simulink model "system_continuous"  (R2026b)
settings: Solver=VariableStepAuto  StopTime=20
values from neighbouring files (symbols this model uses):
  A_sys = zeros(14, 14)    [controller_observer_design.m]    (also in setup.m)
  B_sys = zeros(14, 4)    [controller_observer_design.m]    (also in setup.m)
  C_sys = zeros(6, 14)    [controller_observer_design.m]    (also in setup.m)
  K = lqr(A_sys, B_sys, Q, R)    [controller_observer_design.m]    (also in setup.m)
  omega2u = [k, k, k, k; L*k, 0, -L*k, 0; 0, L*k, 0, -L*k; b, -b, b, -b]    [controller_observer_design.m]    (also in notes.m; setup.m)
  parameters =     [parameters.mat]
  u2omega = (1/(4*b*L*k)) * [b*L, 2*b, 0, L*k; b*L, 0, 2*b, -L*k; b*L, -2*b, 0, L*k; b*L, 0, -2*b, -L*k]    [controller_observer_design.m]    (also in notes.m; setup.m)
undefined symbols (not defined in the file or in its folder): L_obs
settings Model: Creator=elton  LastModifiedBy=elton

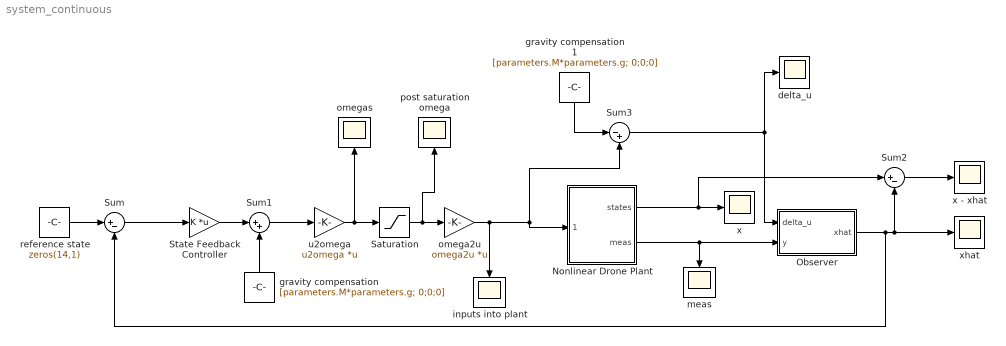
== system system_continuous ==
  Nonlinear Drone Plant : Subsystem
  Observer : Subsystem
  Saturation : Saturate  UpperLimit=250000  LowerLimit=-250000
  State Feedback Controller : Gain  Gain=K  Multiplication=Matrix(K*u)
  Sum : Sum  Inputs=|+-
  Sum1 : Sum  Inputs=|++
  Sum2 : Sum  Inputs=|+-
  Sum3 : Sum  Inputs=|-+
  delta_u : Scope
      settings: ActiveDisplayYMinimum=-0.1401923631580794  ActiveDisplayYMaximum=0.1652403175832419
  gravity compensation : Constant  Value=[parameters.M*parameters.g; 0;0;0]
  gravity compensation1 : Constant  Value=[parameters.M*parameters.g; 0;0;0]
  inputs into plant : Scope
      settings: ActiveDisplayYMinimum=-2.3883084159431922  ActiveDisplayYMaximum=20.39828479264926  DataLoggingVariableName=ScopeData7
  meas : Scope
      settings: ActiveDisplayYMinimum=-955.77756320006051  ActiveDisplayYMaximum=3490.5526217286788
  omega2u : Gain  Gain=omega2u  Multiplication=Matrix(K*u)
  omegas : Scope
      settings: ActiveDisplayYMinimum=-2.059012913011611E+9  ActiveDisplayYMaximum=2.4856689660528789E+9  DataLoggingVariableName=ScopeData8
  post saturation omega : Scope
      settings: ActiveDisplayYMinimum=126867.29383047414  ActiveDisplayYMaximum=168019.94398868005  DataLoggingVariableName=ScopeData9
  reference state : Constant  Value=zeros(14,1)
  u2omega : Gain  Gain=u2omega  Multiplication=Matrix(K*u)
  x : Scope
      settings: ActiveDisplayYMinimum=-2.6435151573110338  ActiveDisplayYMaximum=2.3244072174192603  DataLoggingVariableName=ScopeData6
  x - xhat : Scope
      settings: ActiveDisplayYMinimum=-0.31631682024418123  ActiveDisplayYMaximum=0.17275572014351576  DataLoggingVariableName=ScopeData2
  xhat : Scope
      settings: ActiveDisplayYMinimum=-2.6439782880906106  ActiveDisplayYMaximum=2.3281571087039121  DataLoggingVariableName=ScopeData3
  wires:
  omega2u/1 -> Sum3/2, Nonlinear Drone Plant/1(inputs), inputs into plant/1
  Nonlinear Drone Plant/1(states) -> x/1, Sum2/1
  Sum2/1 -> x - xhat/1
  Sum/1 -> State Feedback Controller/1
  gravity compensation1/1 -> Sum3/1
  reference state/1 -> Sum/1
  gravity compensation/1 -> Sum1/2
  Observer/1(xhat) -> xhat/1, Sum2/2, Sum/2
  u2omega/1 -> Saturation/1, omegas/1
  Saturation/1 -> post saturation omega/1, omega2u/1
  State Feedback Controller/1 -> Sum1/1
  Sum3/1 -> delta_u/1, Observer/1(delta_u)
  Sum1/1 -> u2omega/1
  Nonlinear Drone Plant/2(meas) -> Observer/2(y), meas/1

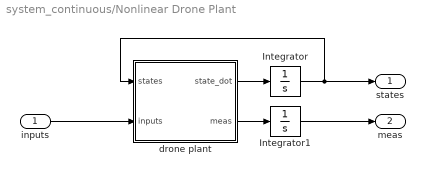
== system system_continuous/Nonlinear Drone Plant ==
  inputs : Inport
  Integrator : Integrator  InitialCondition=[zeros(12,1);0.05;0]
  Integrator1 : Integrator
  drone plant : MATLAB Function  TreatAsAtomicUnit=on
  states : Outport
  meas : Outport  Port=2
  wires:
  drone plant/1(state_dot) -> Integrator/1
  Integrator/1 -> states/1, drone plant/1(states)
  inputs/1 -> drone plant/2(inputs)
  Integrator1/1 -> meas/1
  drone plant/2(meas) -> Integrator1/1

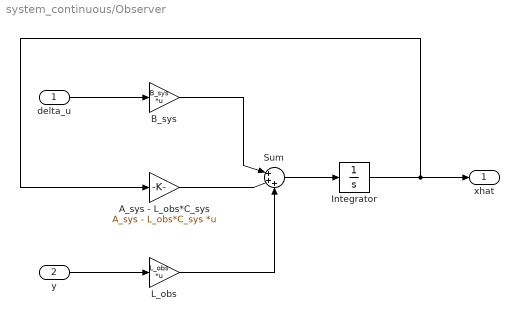
== system system_continuous/Observer ==
  delta_u : Inport
  y : Inport  Port=2
  A_sys - L_obs*C_sys : Gain  Gain=A_sys - L_obs*C_sys  Multiplication=Matrix(K*u)
  B_sys : Gain  Gain=B_sys  Multiplication=Matrix(K*u)
  Integrator : Integrator
  L_obs : Gain  Gain=L_obs  Multiplication=Matrix(K*u)
  Sum : Sum  Inputs=|+++
  xhat : Outport
  wires:
  y/1 -> L_obs/1
  B_sys/1 -> Sum/1
  L_obs/1 -> Sum/3
  A_sys - L_obs*C_sys/1 -> Sum/2
  Sum/1 -> Integrator/1
  Integrator/1 -> A_sys - L_obs*C_sys/1, xhat/1
  delta_u/1 -> B_sys/1

== matlab function system_continuous/Nonlinear Drone Plant/drone plant ==
  data: states input size=14; inputs input size=4; state_dot output size=14; parameters parameter; meas output
%% non-linear state space
function [state_dot, meas]  = nonlin_state_space(states, inputs, parameters)
m     = parameters.m;
m_p    = parameters.m_p;
M     = m + m_p;
g     = parameters.g;
l     = parameters.l;
k_D    = parameters.k_D;
I_xx  = parameters.I_xx;
I_yy  = parameters.I_yy;
I_zz  = parameters.I_zz;

xi = states(1:3);
xi_dot = states(4:6);
eta = states(7:9);
nu = states(10:12);
alpha = states(13);
alpha_dot = states(14);

u_T = inputs(1);
tau = inputs(2:4);

x_dot = xi_dot(1);
y_dot = xi_dot(2);
z_dot = xi_dot(3);

% kinematics
phi = eta(1);
theta = eta(2);
psi = eta(3);
W_inv = [1,  sin(phi)*tan(theta), cos(phi)*tan(theta);
    0,  cos(phi),            -sin(phi);
    0,  sin(phi)/cos(theta), cos(phi)/cos(theta)];

eta_dot = W_inv*nu;

%rotational dynamics
p_dot = (tau(1)/I_xx) + ((I_yy-I_zz)/I_xx)*nu(2)*nu(3);
q_dot = (tau(2)/I_yy) + ((I_zz-I_xx)/I_yy)*nu(1)*nu(3);
r_dot = (tau(3)/I_zz) + ((I_xx-I_yy)/I_zz)*nu(1)*nu(2);
nu_dot = [p_dot; q_dot; r_dot];

%translational dynamics
c_alpha = cos(alpha);
s_alpha = sin(alpha);
c_phi = cos(phi); s_phi = sin(phi);
c_theta = cos(theta); s_theta = sin(theta);
c_psi = cos(psi); s_psi = sin(psi);

Fx = (c_psi*s_theta*c_phi + s_psi*s_phi) * u_T;
Fy = (s_psi*s_theta*c_phi - c_psi*s_phi) * u_T;
Fz = c_theta*c_phi * u_T;

x_dotdot = (1/(m*M)) * ( (m + m_p*c_alpha^2)*(Fx - k_D*x_dot) - m_p*s_alpha*c_alpha*(Fz - k_D*z_dot) + m*m_p*l*alpha_dot^2*s_alpha );
y_dotdot = (Fy - k_D*y_dot) / m;
z_dotdot = (1/(m*M)) * ( (m + m_p*s_alpha^2)*(Fz - k_D*z_dot) - m_p*s_alpha*c_alpha*(Fx - k_D*x_dot) + m*m_p*l*alpha_dot^2*c_alpha ) - g;
xi_dotdot = [x_dotdot; y_dotdot; z_dotdot];

% pendulum dynamics
%alpha_dotdot = (1 / (M * l)) * ( -Fx * c_alpha + Fz * s_alpha + k_D * x_dot * c_alpha - k_D * z_dot * s_alpha );
alpha_dotdot = (1/l)*(-x_dotdot*c_alpha - z_dotdot*s_alpha+g*s_alpha);

% assemble state_dot and meas
state_dot = [xi_dot; xi_dotdot; eta_dot; nu_dot; alpha_dot; alpha_dotdot];
meas = [xi_dot; eta_dot];
end
